simulink model "FeedforwardTest"  (R2026b)
settings: Solver=ode4  StopTime=fixtureCfg.Duration  FixedStep=experimentCfg.Step
PostLoadFcn:
  | addpath(fullfile(fileparts(fileparts(fileparts(fileparts(fileparts(get_param(bdroot,'FileName')))))),'docs','scripts'));initialize_motor_paths();initialize_motor_model(bdroot);
model workspace (MAT data in the model file):
  currentCfg.Ts = 0.0001
  currentCfg.BandwidthHz = 500
  currentCfg.Kpd = 3.14159265359
  currentCfg.Kpq = 3.76991118431
  currentCfg.Kid = 1570.79632679
  currentCfg.Kiq = 1570.79632679
  currentCfg.Kaw = 1000
  deadtimeCfg.DeadTime = 2e-06
  deadtimeCfg.DeviceDrop = 0
  deadtimeCfg.CurrentBlend = 0.1
  deadtimeCfg.ModelEnable = 0
  deadtimeCfg.CompensationEnable = 0
  deadtimeCfg.CompensationScale = 1
  deadtimeCfg.SwitchingStep = 1e-07
  experimentCfg.Step = 5e-06
  experimentCfg.LogTs = 0.0001
  experimentCfg.Duration = 1.5
  experimentCfg.Mode = 2
  experimentCfg.UseInverter = 1
  experimentCfg.UseTiming = 1
  experimentCfg.UseMechanical = 1
  experimentCfg.ImposedElectricalSpeed = 0
  experimentCfg.IdReference = 0
  experimentCfg.IqReference = 2
  experimentCfg.IqInitial = 0
  experimentCfg.SpeedReference = 40
  experimentCfg.SpeedInitial = 0
  experimentCfg.PositionReference = 1
  experimentCfg.PositionInitial = 0
  experimentCfg.CommandTime = 0.05
  experimentCfg.LoadTorque = 0.1
  experimentCfg.LoadTime = 0.35
  experimentCfg.Enable = 1
  experimentCfg.Reset = 0
  feedforwardCfg.Enable = 1
  feedforwardCfg.ParameterScale = 1
  fixtureCfg.Ts = 0.0001
  fixtureCfg.Duration = 0.03
  fixtureCfg.SolverStep = 5e-06
  fixtureCfg.Id = 1
  fixtureCfg.Iq = 2
  fixtureCfg.ElectricalSpeed = 1000
  fixtureCfg.Enable = 1
  fixtureCfg.Inputs = [1 1 1 1 1 1 1 1 1 1 1 1 ... (903 elements, 301x3)]
  inverterCfg.Vdc = 48
  inverterCfg.MinDuty = 0.02
  inverterCfg.PwmTs = 0.0001
  inverterCfg.LinearLimit = 26.6043004043
  motionCfg.Ts = 0.001
  motionCfg.NaturalFrequency = 20
  motionCfg.Damping = 0.9
  motionCfg.Kt = 0.21
  motionCfg.Kp = 0.0852380952381
  motionCfg.Ki = 0.952380952381
  motionCfg.Kaw = 20
  motionCfg.PositionKp = 8
  motionCfg.SpeedLimit = 80
  motionCfg.AccelerationLimit = 200
  motionCfg.CurrentLimit = 8
  pmsmCfg.Rs = 0.5
  pmsmCfg.Ld = 0.001
  pmsmCfg.Lq = 0.0012
  pmsmCfg.Flux = 0.035
  pmsmCfg.PolePairs = 4
  pmsmCfg.J = 0.0005
  pmsmCfg.B = 0.0001
  pmsmCfg.Id0 = 0
  pmsmCfg.Iq0 = 0
  pmsmCfg.Speed0 = 0
  pmsmCfg.Position0 = 0
  testStim.time = []
  testStim.signals.values = [1 1 1 1 1 1 1 1 1 1 1 1 ... (903 elements, 301x3)]
  testStim.signals.dimensions = 3
  timingCfg.Ts = 0.0001
  timingCfg.FeedbackTicks = 1
  timingCfg.ActuationTicks = 1
libraries: DQFeedforward x1
settings Model: Creator=24322  LastModifiedBy=24322

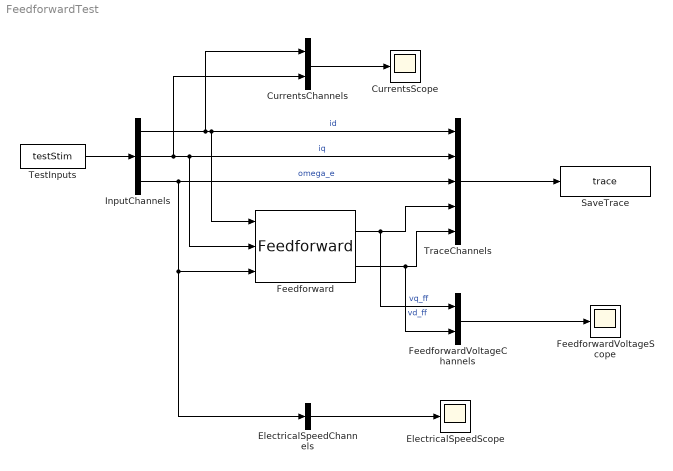
== system FeedforwardTest ==
  CurrentsChannels : Mux  Inputs=2
  CurrentsScope : Scope
      settings: Title=Currents  YLabel=A
  ElectricalSpeedChannels : Mux  Inputs=1
  ElectricalSpeedScope : Scope
      settings: Title=ElectricalSpeed  YLabel=rad/s
  Feedforward : DQFeedforward/Feedforward  SystemSampleTime=-1  VariantActivationTime=update diagram  EmptyChoice=off  PassThrough=off  PassThroughVariantControl=(default)  EmptyChoiceVariantControl=(default)  AllowFlexibleInterface=on  Latency=0  AutoFrameSizeCalculation=off
  FeedforwardVoltageChannels : Mux  Inputs=2
  FeedforwardVoltageScope : Scope
      settings: Title=FeedforwardVoltage  YLabel=V
  InputChannels : Demux  Outputs=3
  SaveTrace : ToWorkspace  VariableName=trace  SaveFormat=Structure With Time  SampleTime=experimentCfg.LogTs
  TestInputs : FromWorkspace  VariableName=testStim  SampleTime=currentCfg.Ts  Interpolate=off  OutputAfterFinalValue=Holding final value
  TraceChannels : Mux  Inputs=5
  wires:
  FeedforwardVoltageChannels/1 -> FeedforwardVoltageScope/1
  ElectricalSpeedChannels/1 -> ElectricalSpeedScope/1
  CurrentsChannels/1 -> CurrentsScope/1
  Feedforward/2 -> FeedforwardVoltageChannels/2, TraceChannels/5  "vq_ff"
  Feedforward/1 -> TraceChannels/4, FeedforwardVoltageChannels/1  "vd_ff"
  TraceChannels/1 -> SaveTrace/1
  InputChannels/3 -> Feedforward/3, ElectricalSpeedChannels/1, TraceChannels/3  "omega_e"
  InputChannels/2 -> Feedforward/2, TraceChannels/2, CurrentsChannels/2  "iq"
  InputChannels/1 -> TraceChannels/1, Feedforward/1, CurrentsChannels/1  "id"
  TestInputs/1 -> InputChannels/1
